simulink model "elec_ss"  (R2023a)
settings: Solver=VariableStepAuto  StartTime=0.0  StopTime=10  RelTol=1e-3
settings Model: Creator=ahmad  LastModifiedBy=ahmad

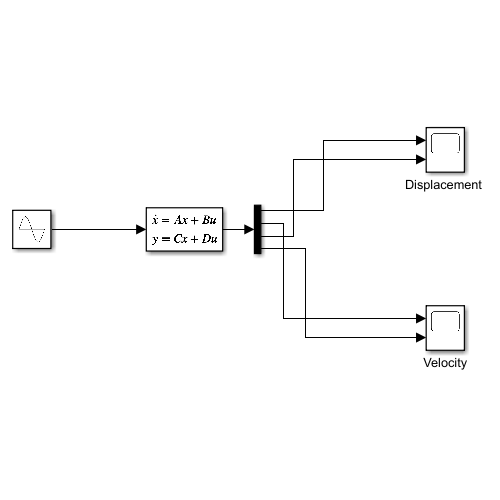
[thumbnail: Simulink's stored preview of the top-level diagram]
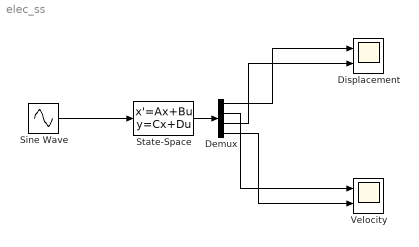
== system elec_ss ==
  Demux : Demux
  "Displacement " : Scope  NumInputPorts=2
  Sine Wave : Sin  Amplitude=5000  Frequency=8*pi  SampleTime=0
  State-Space : StateSpace  A=|  B=[0; 0.00025; 0; 0]  C=[1, 0, 0, 0;0, 1, 0, 0; 0, 0, 1, 0;0, 0, 0, 1];  D=[0;0;0;0]  InitialCondition=[0 0 0 0]
      | [ 0 1 0 0;
      |  -1100 -1500 50 500;
      |   0 0 0 1;
      |  1000 10000 -1000 -10000 ]
  Velocity : Scope  NumInputPorts=2
  wires:
  Demux/2 -> Velocity/1
  Demux/1 -> "Displacement "/1
  Demux/4 -> Velocity/2
  Sine Wave/1 -> State-Space/1
  State-Space/1 -> Demux/1
  Demux/3 -> "Displacement "/2
